simulink model "sixswitch"  (R2024b)
settings: Solver=ode23tb  StartTime=0.0  StopTime=1.0  MaxStep=sixswitch_maxstep  RelTol=1e-4
InitFcn:
  | p2s_dir = fileparts(get_param(bdroot, 'FileName'));
  | if ~isempty(p2s_dir), addpath(p2s_dir); end
  | clear p2s_dir
  | sixswitch_params;
values from neighbouring files (symbols this model uses):
  decouple_gain = 2*pi*fgrid*L    (= 0.125663706144)    [sixswitch_params.m]
  fgrid = 50    [sixswitch_params.m]
  fs = 100e3    (= 100000)    [sixswitch_params.m]
  grid_sr = 32e3    (= 32000)    [sixswitch_params.m]
  gridFrequency = 50    [sixswitch_params.m]
  id_ref_const = 13.8    [sixswitch_params.m]
  load_ramp_X0 = 100    [sixswitch_params.m]
  load_ramp_XFinal = 18000    [sixswitch_params.m]
  Pss = struct()    [sixswitch_params.m]
  vc_avg_T = (1/fs)*10    (= 0.0001)    [sixswitch_params.m]
  vd_dec_const = -10    [sixswitch_params.m]
  Vdc_ref = Vin    (= 700)    [sixswitch_params.m]
  Vgrid_pk = (gridVoltageLLrms/sqrt(3))*sqrt(2)    [sixswitch_params.m]
  vq_const = -1.85    [sixswitch_params.m]
undefined symbols (not defined in the file or in its folder): cc, pll, sixswitch_y0, vc
libraries: slpidlib x4
Description:
  | Ideal-switch translation of SixSwitch.plecs (see README.md)
settings Model: Creator=Jonathan  LastModifiedBy=Jonathan
settings SolverCC: ZeroCrossAlgorithm=Adaptive
settings DebuggingCC: MaxConsecutiveZCsMsg=none

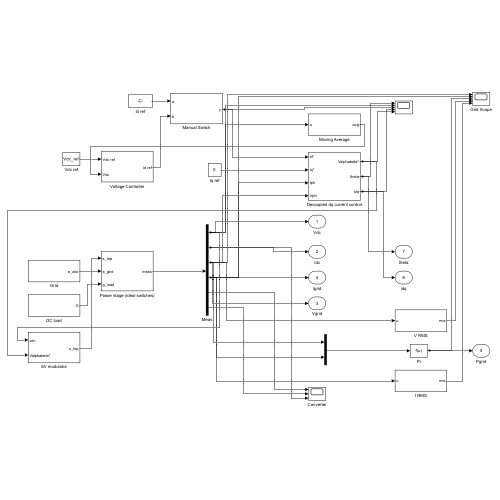
[thumbnail: Simulink's stored preview of the top-level diagram]
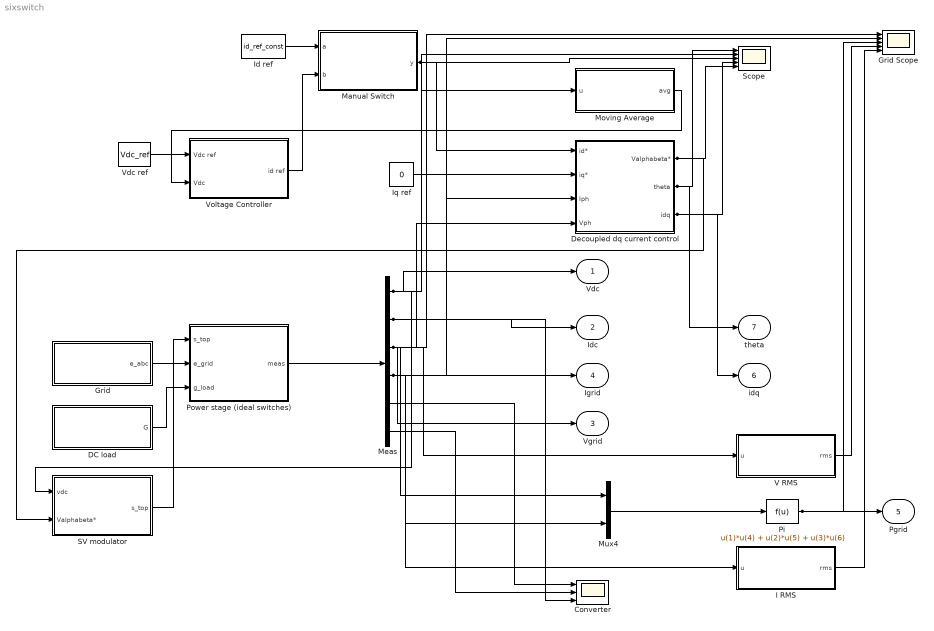
== system sixswitch ==
  Converter : Scope  NumInputPorts=3
  DC load : Subsystem
  Decoupled dq current control : Subsystem
  Grid : Subsystem
  Grid Scope : Scope  NumInputPorts=5
  I RMS : Subsystem
  Id ref : Constant  Value=id_ref_const
  Iq ref : Constant  Value=0
  Manual Switch : Subsystem
  Meas : Demux  Outputs=[1 1 3 3 3 3]
  Moving Average : Subsystem
  Mux4 : Mux  Inputs=2
  Pi : Fcn  Expr=u(1)*u(4) + u(2)*u(5) + u(3)*u(6)
  Power stage (ideal switches) : Subsystem
  SV modulator : Subsystem
  Scope : Scope  NumInputPorts=5
  V RMS : Subsystem
  Vdc ref : Constant  Value=Vdc_ref
  Voltage Controller : Subsystem
  Vdc : Outport
  Idc : Outport  Port=2
  Vgrid : Outport  Port=3
  Igrid : Outport  Port=4
  Pgrid : Outport  Port=5
  idq : Outport  Port=6
  theta : Outport  Port=7
  wires:
  Id ref/1 -> Manual Switch/1(a)
  Vdc ref/1 -> Voltage Controller/1(Vdc ref)
  Grid/1(e_abc) -> Power stage (ideal switches)/2(e_grid)
  DC load/1(G) -> Power stage (ideal switches)/3(g_load)
  Voltage Controller/1(id ref) -> Manual Switch/2(b)
  SV modulator/1(s_top) -> Power stage (ideal switches)/1(s_top)
  Power stage (ideal switches)/1(meas) -> Meas/1
  Manual Switch/1(y) -> Scope/3, Decoupled dq current control/1(id*)
  Iq ref/1 -> Decoupled dq current control/2(iq*)
  Decoupled dq current control/2(theta) -> Scope/1, theta/1
  Decoupled dq current control/1(Valphabeta*) -> SV modulator/2(Valphabeta*), Scope/5
  Meas/2 -> Converter/3, Idc/1
  Meas/1 -> Scope/2, Moving Average/1(u), SV modulator/1(vdc), Vdc/1
  Meas/3 -> V RMS/1(u), Decoupled dq current control/4(Vph), Mux4/1, Grid Scope/1, Vgrid/1
  Meas/4 -> Grid Scope/2, I RMS/1(u), Decoupled dq current control/3(Iph), Mux4/2, Igrid/1
  Meas/5 -> Converter/1
  Meas/6 -> Converter/2
  Moving Average/1(avg) -> Voltage Controller/2(Vdc)
  Decoupled dq current control/3(idq) -> Scope/4, idq/1
  Mux4/1 -> Pi/1
  V RMS/1(rms) -> Grid Scope/4
  Pi/1 -> Grid Scope/3, Pgrid/1
  I RMS/1(rms) -> Grid Scope/5

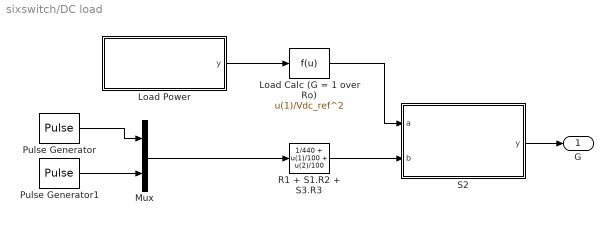
== system sixswitch/DC load ==
  Load Calc (G = 1 over Ro) : Fcn  Expr=u(1)/Vdc_ref^2
  Load Power : Subsystem
  Mux : Mux  Inputs=2
  Pulse Generator : DiscretePulseGenerator  PulseType=Time based  Period=0.02  PulseWidth=50  PhaseDelay=0.030
  Pulse Generator1 : DiscretePulseGenerator  PulseType=Time based  Period=0.01  PulseWidth=50  PhaseDelay=0.045
  R1 + S1.R2 + S3.R3 : Fcn  Expr=1/440 + u(1)/100 + u(2)/100
  S2 : Subsystem
  G : Outport
  wires:
  R1 + S1.R2 + S3.R3/1 -> S2/2(b)
  Mux/1 -> R1 + S1.R2 + S3.R3/1
  Pulse Generator/1 -> Mux/1
  Pulse Generator1/1 -> Mux/2
  Load Power/1(y) -> Load Calc (G = 1 over Ro)/1
  Load Calc (G = 1 over Ro)/1 -> S2/1(a)
  S2/1(y) -> G/1

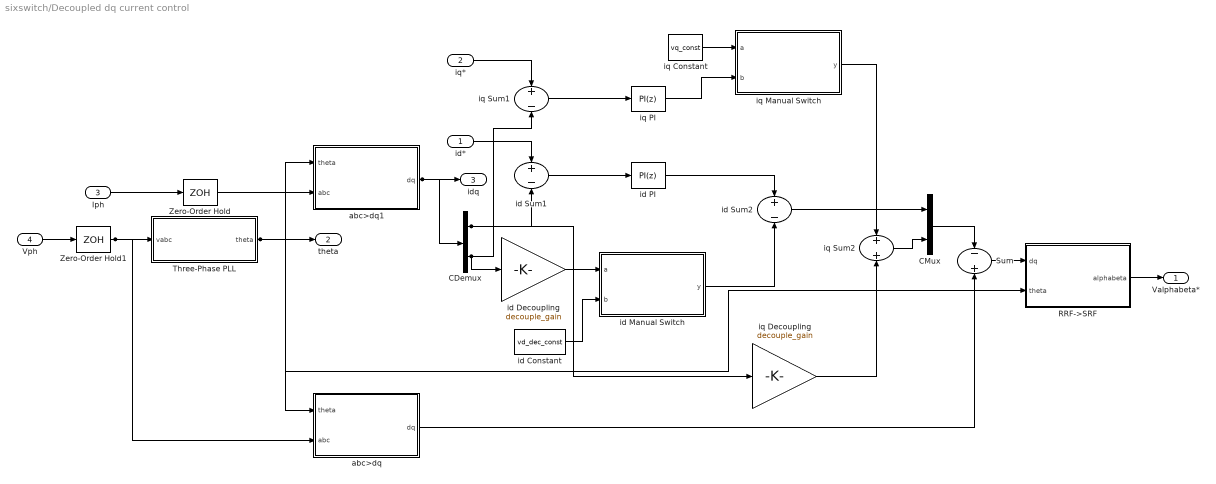
== system sixswitch/Decoupled dq current control ==
  id* : Inport
  iq* : Inport  Port=2
  Iph : Inport  Port=3
  Vph : Inport  Port=4
  CDemux : Demux  Outputs=2
  CMux : Mux  Inputs=2
  RRF->SRF : Subsystem
  Sum : Sum  Inputs=-+
  Three-Phase PLL : Subsystem
  Zero-Order Hold : ZeroOrderHold  SampleTime=1/grid_sr
  Zero-Order Hold1 : ZeroOrderHold  SampleTime=1/grid_sr
  abc>dq : Subsystem
  abc>dq1 : Subsystem
  id Constant : Constant  Value=vd_dec_const
  id Decoupling : Gain  Gain=decouple_gain
  id Manual Switch : Subsystem
  id PI : slpidlib/PID Controller  Controller=PI  Form=Parallel  TimeDomain=Discrete-time  UseExternalTs=off  SampleTime=cc.Ts  IntegratorMethod=Forward Euler  FilterMethod=Forward Euler  ControllerParametersSource=internal  P=cc.kp  I=cc.ki  UseKiTs=off  D=0  UseExternalDerivativeSource=off  N=100  UseFilter=on  TunerSelectOption=Transfer Function Based (PID Tuner App)  InitialConditionSource=internal  InitialConditionForIntegrator=0  InitialConditionForFilter=0  DifferentiatorICPrevScaledInput=0  ExternalReset=none  TrackingMode=off  Kt=1  LimitOutput=on  SatLimitsSource=internal  UpperSaturationLimit=cc.up  LowerSaturationLimit=cc.lo  LinearizeAsGain=off  AntiWindupMode=clamping  Kb=1  LimitIntegrator=off  UpperIntegratorSaturationLimit=inf  LowerIntegratorSaturationLimit=-inf  POutMin=[]  POutMax=[]  IOutMin=[]  IOutMax=[]  DOutMin=[]  DOutMax=[]  NOutMin=[]  NOutMax=[]  SumOutMin=[]  SumOutMax=[]  SaturationOutMin=[]  SaturationOutMax=[]  PParamMin=[]  PParamMax=[]  IParamMin=[]  IParamMax=[]  DParamMin=[]  DParamMax=[]  NParamMin=[]  NParamMax=[]  KbParamMin=[]  KbParamMax=[]  KtParamMin=[]  KtParamMax=[]  KbOutMin=[]  KbOutMax=[]  KtOutMin=[]  KtOutMax=[]  IntegratorOutMin=[]  IntegratorOutMax=[]  FilterOutMin=[]  FilterOutMax=[]  SumI1OutMin=[]  SumI1OutMax=[]  SumI2OutMin=[]  SumI2OutMax=[]  SumI3OutMin=[]  SumI3OutMax=[]  SumI4OutMin=[]  SumI4OutMax=[]  SumDOutMin=[]  SumDOutMax=[]  DifferentiatorOutMin=[]  DifferentiatorOutMax=[]  FilterDiffOutCoefMin=[]  FilterDiffOutCoefMax=[]  ReciprocalOutMin=[]  ReciprocalOutMax=[]  SumDenOutMin=[]  SumDenOutMax=[]  SumNumOutMin=[]  SumNumOutMax=[]  DivideOutMin=[]  DivideOutMax=[]  UdiffTsProdOutMin=[]  UdiffTsProdOutMax=[]  NTsProdOutMin=[]  NTsProdOutMax=[]  UintegralTsProdOutMin=[]  UintegralTsProdOutMax=[]  UngainTsProdOutMin=[]  UngainTsProdOutMax=[]  ClampingZeroOutDataTypeStr=Inherit: Inherit via back propagation  ClampingZeroOutMin=[]  ClampingZeroOutMax=[]  FilterDenConstantOutDataTypeStr=Inherit: Inherit via back propagation  FilterDenConstantOutMin=[]  FilterDenConstantOutMax=[]  PCopyOutDataTypeStr=Inherit: Inherit via back propagation  PCopyOutMin=[]  PCopyOutMax=[]  NCopyOutDataTypeStr=Inherit: Inherit via back propagation  NCopyOutMin=[]  NCopyOutMax=[]  IntegratorContinuousStateAttributes=''  IntegratorStateMustResolveToSignalObject=off  IntegratorRTWStateStorageClass=Auto  FilterContinuousStateAttributes=''  FilterStateMustResolveToSignalObject=off  FilterRTWStateStorageClass=Auto  ParallelPVariant=InternalParameters  IdealPVariant=Disabled  IVariant=InternalParameters  DVariant=Disabled  IntegratorVariant=Discrete  SatVariant=Enabled  AWVariant=DiscClampingParallel  PCopyVariant=Disabled  TRVariant=Disabled  FdbkBlocksVariant=Forward  IdealPFdbkVariant=Disabled  SatFdbkVariant=Disabled  DerivativeFilterVariant=Disabled  NVariant=Disabled  NCopyVariant=Disabled_SignalSpec  FilterICVariant=Disabled  IntegratorICVariant=InternalICs  ExternalResetVariant=Disabled  TRSumVariant=Passthrough  SumFdbkVariant=Disabled  SumVariant=Sum_PI  TsampFilterVariant=InternalTs  TsampNgainVariant=Passthrough  TsampIntegralVariant=Disabled_SignalSpec  ExternalSaturationOutDataTypeStr=Inherit: Same as second input  DerivativeSourceVariant=Disabled  PreIntVariant=InternalPreInt
      settings: LibrarySourceBlock=simulink/Discrete/Discrete PID Controller
  id Sum1 : Sum  Inputs=+-
  id Sum2 : Sum  Inputs=+-
  iq Constant : Constant  Value=vq_const
  iq Decoupling : Gain  Gain=decouple_gain
  iq Manual Switch : Subsystem
  iq PI : slpidlib/PID Controller  Controller=PI  Form=Parallel  TimeDomain=Discrete-time  UseExternalTs=off  SampleTime=cc.Ts  IntegratorMethod=Forward Euler  FilterMethod=Forward Euler  ControllerParametersSource=internal  P=cc.kp  I=cc.ki  UseKiTs=off  D=0  UseExternalDerivativeSource=off  N=100  UseFilter=on  TunerSelectOption=Transfer Function Based (PID Tuner App)  InitialConditionSource=internal  InitialConditionForIntegrator=0  InitialConditionForFilter=0  DifferentiatorICPrevScaledInput=0  ExternalReset=none  TrackingMode=off  Kt=1  LimitOutput=on  SatLimitsSource=internal  UpperSaturationLimit=cc.up  LowerSaturationLimit=cc.lo  LinearizeAsGain=off  AntiWindupMode=back-calculation  Kb=cc.kbc  LimitIntegrator=off  UpperIntegratorSaturationLimit=inf  LowerIntegratorSaturationLimit=-inf  POutMin=[]  POutMax=[]  IOutMin=[]  IOutMax=[]  DOutMin=[]  DOutMax=[]  NOutMin=[]  NOutMax=[]  SumOutMin=[]  SumOutMax=[]  SaturationOutMin=[]  SaturationOutMax=[]  PParamMin=[]  PParamMax=[]  IParamMin=[]  IParamMax=[]  DParamMin=[]  DParamMax=[]  NParamMin=[]  NParamMax=[]  KbParamMin=[]  KbParamMax=[]  KtParamMin=[]  KtParamMax=[]  KbOutMin=[]  KbOutMax=[]  KtOutMin=[]  KtOutMax=[]  IntegratorOutMin=[]  IntegratorOutMax=[]  FilterOutMin=[]  FilterOutMax=[]  SumI1OutMin=[]  SumI1OutMax=[]  SumI2OutMin=[]  SumI2OutMax=[]  SumI3OutMin=[]  SumI3OutMax=[]  SumI4OutMin=[]  SumI4OutMax=[]  SumDOutMin=[]  SumDOutMax=[]  DifferentiatorOutMin=[]  DifferentiatorOutMax=[]  FilterDiffOutCoefMin=[]  FilterDiffOutCoefMax=[]  ReciprocalOutMin=[]  ReciprocalOutMax=[]  SumDenOutMin=[]  SumDenOutMax=[]  SumNumOutMin=[]  SumNumOutMax=[]  DivideOutMin=[]  DivideOutMax=[]  UdiffTsProdOutMin=[]  UdiffTsProdOutMax=[]  NTsProdOutMin=[]  NTsProdOutMax=[]  UintegralTsProdOutMin=[]  UintegralTsProdOutMax=[]  UngainTsProdOutMin=[]  UngainTsProdOutMax=[]  ClampingZeroOutDataTypeStr=Inherit: Inherit via back propagation  ClampingZeroOutMin=[]  ClampingZeroOutMax=[]  FilterDenConstantOutDataTypeStr=Inherit: Inherit via back propagation  FilterDenConstantOutMin=[]  FilterDenConstantOutMax=[]  PCopyOutDataTypeStr=Inherit: Inherit via back propagation  PCopyOutMin=[]  PCopyOutMax=[]  NCopyOutDataTypeStr=Inherit: Inherit via back propagation  NCopyOutMin=[]  NCopyOutMax=[]  IntegratorContinuousStateAttributes=''  IntegratorStateMustResolveToSignalObject=off  IntegratorRTWStateStorageClass=Auto  FilterContinuousStateAttributes=''  FilterStateMustResolveToSignalObject=off  FilterRTWStateStorageClass=Auto  ParallelPVariant=InternalParameters  IdealPVariant=Disabled  IVariant=InternalParameters  DVariant=Disabled  IntegratorVariant=Discrete  SatVariant=Enabled  AWVariant=BackCalculation  PCopyVariant=Disabled  TRVariant=Disabled  FdbkBlocksVariant=Forward  IdealPFdbkVariant=Disabled  SatFdbkVariant=Disabled  DerivativeFilterVariant=Disabled  NVariant=Disabled  NCopyVariant=Disabled_SignalSpec  FilterICVariant=Disabled  IntegratorICVariant=InternalICs  ExternalResetVariant=Disabled  TRSumVariant=Passthrough  SumFdbkVariant=Disabled  SumVariant=Sum_PI  TsampFilterVariant=InternalTs  TsampNgainVariant=Passthrough  TsampIntegralVariant=Disabled_SignalSpec  ExternalSaturationOutDataTypeStr=Inherit: Same as second input  DerivativeSourceVariant=Disabled  PreIntVariant=InternalPreInt
      settings: LibrarySourceBlock=simulink/Discrete/Discrete PID Controller
  iq Sum1 : Sum  Inputs=+-
  iq Sum2 : Sum
  Valphabeta* : Outport
  theta : Outport  Port=2
  idq : Outport  Port=3
  wires:
  Vph/1 -> Zero-Order Hold1/1
  Iph/1 -> Zero-Order Hold/1
  Zero-Order Hold1/1 -> abc>dq/2(abc), Three-Phase PLL/1(vabc)
  CMux/1 -> Sum/1
  Zero-Order Hold/1 -> abc>dq1/2(abc)
  id Manual Switch/1(y) -> id Sum2/2
  iq*/1 -> iq Sum1/1
  Three-Phase PLL/1(theta) -> RRF->SRF/2(theta), abc>dq1/1(theta), theta/1, abc>dq/1(theta)
  abc>dq1/1(dq) -> CDemux/1, idq/1
  RRF->SRF/1(alphabeta) -> Valphabeta*/1
  abc>dq/1(dq) -> Sum/2
  id Constant/1 -> id Manual Switch/2(b)
  id Decoupling/1 -> id Manual Switch/1(a)
  id*/1 -> id Sum1/1
  CDemux/1 -> id Sum1/2, iq Decoupling/1
  id PI/1 -> id Sum2/1
  CDemux/2 -> iq Sum1/2, id Decoupling/1
  iq Sum1/1 -> iq PI/1
  id Sum1/1 -> id PI/1
  iq Decoupling/1 -> iq Sum2/2
  iq Constant/1 -> iq Manual Switch/1(a)
  iq PI/1 -> iq Manual Switch/2(b)
  iq Manual Switch/1(y) -> iq Sum2/1
  id Sum2/1 -> CMux/1
  iq Sum2/1 -> CMux/2
  Sum/1 -> RRF->SRF/1(dq)

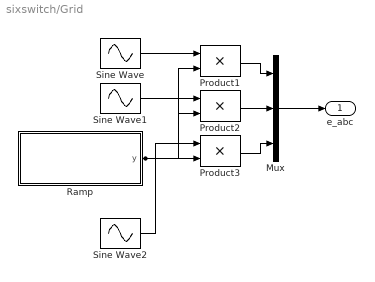
== system sixswitch/Grid ==
  Mux : Mux  Inputs=3
  Product1 : Product  Inputs=**
  Product2 : Product  Inputs=**
  Product3 : Product  Inputs=**
  Ramp : Subsystem
  Sine Wave : Sin  Amplitude=Vgrid_pk  Frequency=2*pi*gridFrequency  SampleTime=0
  Sine Wave1 : Sin  Amplitude=Vgrid_pk  Frequency=2*pi*gridFrequency  Phase=-2*pi/3  SampleTime=0
  Sine Wave2 : Sin  Amplitude=Vgrid_pk  Frequency=2*pi*gridFrequency  Phase=2*pi/3  SampleTime=0
  e_abc : Outport
  wires:
  Sine Wave/1 -> Product1/1
  Sine Wave1/1 -> Product2/1
  Product1/1 -> Mux/1
  Sine Wave2/1 -> Product3/1
  Ramp/1(y) -> Product1/2, Product2/2, Product3/2
  Product2/1 -> Mux/2
  Product3/1 -> Mux/3
  Mux/1 -> e_abc/1

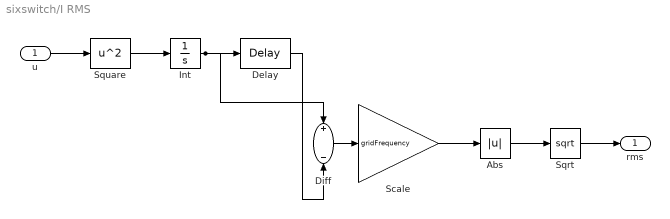
== system sixswitch/I RMS ==
  u : Inport
  Abs : Abs  SaturateOnIntegerOverflow=off
  Delay : TransportDelay  DelayTime=1/(gridFrequency)  BufferSize=131072
  Diff : Sum  Inputs=+-
  Int : Integrator
  Scale : Gain  Gain=gridFrequency
  Sqrt : Sqrt
  Square : Math  Operator=square
  rms : Outport
  wires:
  u/1 -> Square/1
  Int/1 -> Diff/1, Delay/1
  Square/1 -> Int/1
  Diff/1 -> Scale/1
  Delay/1 -> Diff/2
  Sqrt/1 -> rms/1
  Abs/1 -> Sqrt/1
  Scale/1 -> Abs/1

== system sixswitch/Manual Switch ==
  a : Inport
  b : Inport  Port=2
  Switch : Switch  Criteria=u2 > Threshold  Threshold=0.5  SaturateOnIntegerOverflow=off  InputSameDT=off
  sel : Constant  Value=double(sel_idref == 1)
  y : Outport
  wires:
  a/1 -> Switch/1
  sel/1 -> Switch/2
  b/1 -> Switch/3
  Switch/1 -> y/1

== system sixswitch/Moving Average ==
  u : Inport
  Delay : TransportDelay  DelayTime=vc_avg_T  BufferSize=131072
  Diff : Sum  Inputs=+-
  Int : Integrator
  Scale : Gain  Gain=1/(vc_avg_T)
  avg : Outport
  wires:
  u/1 -> Int/1
  Int/1 -> Diff/1, Delay/1
  Delay/1 -> Diff/2
  Scale/1 -> avg/1
  Diff/1 -> Scale/1

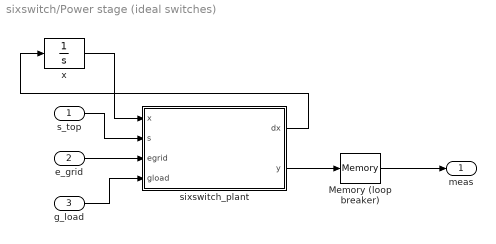
== system sixswitch/Power stage (ideal switches) ==
  s_top : Inport
  e_grid : Inport  Port=2
  g_load : Inport  Port=3
  Memory (loop breaker) : Memory  InitialCondition=sixswitch_y0
  sixswitch_plant : MATLAB Function  TreatAsAtomicUnit=on
  x : Integrator  InitialCondition=Pss.x0
  meas : Outport
  wires:
  x/1 -> sixswitch_plant/1(x)
  sixswitch_plant/2(y) -> Memory (loop breaker)/1
  sixswitch_plant/1(dx) -> x/1
  s_top/1 -> sixswitch_plant/2(s)
  e_grid/1 -> sixswitch_plant/3(egrid)
  g_load/1 -> sixswitch_plant/4(gload)
  Memory (loop breaker)/1 -> meas/1

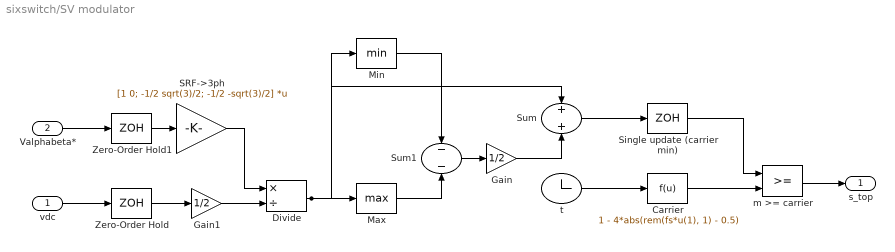
== system sixswitch/SV modulator ==
  vdc : Inport
  Valphabeta* : Inport  Port=2
  Carrier : Fcn  Expr=1 - 4*abs(rem(fs*u(1), 1) - 0.5)
  Divide : Product  Inputs=*/
  Gain : Gain  Gain=1/2
  Gain1 : Gain  Gain=1/2
  Max : MinMax  Function=max
  Min : MinMax
  SRF->3ph : Gain  Gain=[1 0; -1/2 sqrt(3)/2; -1/2 -sqrt(3)/2]  Multiplication=Matrix(K*u)
  Single update (carrier min) : ZeroOrderHold  SampleTime=1/fs
  Sum : Sum
  Sum1 : Sum  Inputs=--
  Zero-Order Hold : ZeroOrderHold  SampleTime=1/fs
  Zero-Order Hold1 : ZeroOrderHold  SampleTime=1/fs
  m >= carrier : RelationalOperator  OutDataTypeStr=boolean  RndMeth=Simplest  InputSameDT=off
  t : Clock
  s_top : Outport
  wires:
  vdc/1 -> Zero-Order Hold/1
  Valphabeta*/1 -> Zero-Order Hold1/1
  Zero-Order Hold/1 -> Gain1/1
  Zero-Order Hold1/1 -> SRF->3ph/1
  Gain1/1 -> Divide/2
  SRF->3ph/1 -> Divide/1
  Divide/1 -> Sum/1, Min/1, Max/1
  Min/1 -> Sum1/1
  Sum1/1 -> Gain/1
  Max/1 -> Sum1/2
  Sum/1 -> Single update (carrier min)/1
  Gain/1 -> Sum/2
  t/1 -> Carrier/1
  Single update (carrier min)/1 -> m >= carrier/1
  Carrier/1 -> m >= carrier/2
  m >= carrier/1 -> s_top/1

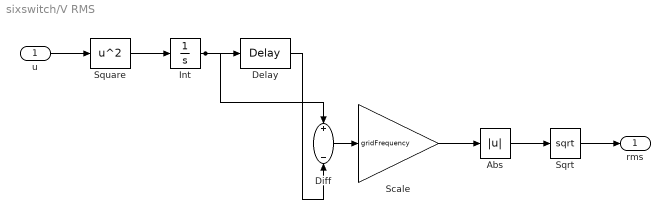
== system sixswitch/V RMS ==
  u : Inport
  Abs : Abs  SaturateOnIntegerOverflow=off
  Delay : TransportDelay  DelayTime=1/(gridFrequency)  BufferSize=131072
  Diff : Sum  Inputs=+-
  Int : Integrator
  Scale : Gain  Gain=gridFrequency
  Sqrt : Sqrt
  Square : Math  Operator=square
  rms : Outport
  wires:
  Square/1 -> Int/1
  u/1 -> Square/1
  Diff/1 -> Scale/1
  Delay/1 -> Diff/2
  Int/1 -> Diff/1, Delay/1
  Abs/1 -> Sqrt/1
  Scale/1 -> Abs/1
  Sqrt/1 -> rms/1

== system sixswitch/Voltage Controller ==
  Vdc ref : Inport
  Vdc : Inport  Port=2
  Discrete PID Controller : slpidlib/PID Controller  Controller=PI  Form=Parallel  TimeDomain=Discrete-time  UseExternalTs=off  SampleTime=vc.Ts  IntegratorMethod=Forward Euler  FilterMethod=Forward Euler  ControllerParametersSource=internal  P=vc.kp  I=vc.ki  UseKiTs=off  D=0  UseExternalDerivativeSource=off  N=100  UseFilter=on  TunerSelectOption=Transfer Function Based (PID Tuner App)  InitialConditionSource=internal  InitialConditionForIntegrator=0  InitialConditionForFilter=0  DifferentiatorICPrevScaledInput=0  ExternalReset=none  TrackingMode=off  Kt=1  LimitOutput=on  SatLimitsSource=internal  UpperSaturationLimit=vc.up  LowerSaturationLimit=vc.lo  LinearizeAsGain=off  AntiWindupMode=clamping  Kb=1  LimitIntegrator=off  UpperIntegratorSaturationLimit=inf  LowerIntegratorSaturationLimit=-inf  POutMin=[]  POutMax=[]  IOutMin=[]  IOutMax=[]  DOutMin=[]  DOutMax=[]  NOutMin=[]  NOutMax=[]  SumOutMin=[]  SumOutMax=[]  SaturationOutMin=[]  SaturationOutMax=[]  PParamMin=[]  PParamMax=[]  IParamMin=[]  IParamMax=[]  DParamMin=[]  DParamMax=[]  NParamMin=[]  NParamMax=[]  KbParamMin=[]  KbParamMax=[]  KtParamMin=[]  KtParamMax=[]  KbOutMin=[]  KbOutMax=[]  KtOutMin=[]  KtOutMax=[]  IntegratorOutMin=[]  IntegratorOutMax=[]  FilterOutMin=[]  FilterOutMax=[]  SumI1OutMin=[]  SumI1OutMax=[]  SumI2OutMin=[]  SumI2OutMax=[]  SumI3OutMin=[]  SumI3OutMax=[]  SumI4OutMin=[]  SumI4OutMax=[]  SumDOutMin=[]  SumDOutMax=[]  DifferentiatorOutMin=[]  DifferentiatorOutMax=[]  FilterDiffOutCoefMin=[]  FilterDiffOutCoefMax=[]  ReciprocalOutMin=[]  ReciprocalOutMax=[]  SumDenOutMin=[]  SumDenOutMax=[]  SumNumOutMin=[]  SumNumOutMax=[]  DivideOutMin=[]  DivideOutMax=[]  UdiffTsProdOutMin=[]  UdiffTsProdOutMax=[]  NTsProdOutMin=[]  NTsProdOutMax=[]  UintegralTsProdOutMin=[]  UintegralTsProdOutMax=[]  UngainTsProdOutMin=[]  UngainTsProdOutMax=[]  ClampingZeroOutDataTypeStr=Inherit: Inherit via back propagation  ClampingZeroOutMin=[]  ClampingZeroOutMax=[]  FilterDenConstantOutDataTypeStr=Inherit: Inherit via back propagation  FilterDenConstantOutMin=[]  FilterDenConstantOutMax=[]  PCopyOutDataTypeStr=Inherit: Inherit via back propagation  PCopyOutMin=[]  PCopyOutMax=[]  NCopyOutDataTypeStr=Inherit: Inherit via back propagation  NCopyOutMin=[]  NCopyOutMax=[]  IntegratorContinuousStateAttributes=''  IntegratorStateMustResolveToSignalObject=off  IntegratorRTWStateStorageClass=Auto  FilterContinuousStateAttributes=''  FilterStateMustResolveToSignalObject=off  FilterRTWStateStorageClass=Auto  ParallelPVariant=InternalParameters  IdealPVariant=Disabled  IVariant=InternalParameters  DVariant=Disabled  IntegratorVariant=Discrete  SatVariant=Enabled  AWVariant=DiscClampingParallel  PCopyVariant=Disabled  TRVariant=Disabled  FdbkBlocksVariant=Forward  IdealPFdbkVariant=Disabled  SatFdbkVariant=Disabled  DerivativeFilterVariant=Disabled  NVariant=Disabled  NCopyVariant=Disabled_SignalSpec  FilterICVariant=Disabled  IntegratorICVariant=InternalICs  ExternalResetVariant=Disabled  TRSumVariant=Passthrough  SumFdbkVariant=Disabled  SumVariant=Sum_PI  TsampFilterVariant=InternalTs  TsampNgainVariant=Passthrough  TsampIntegralVariant=Disabled_SignalSpec  ExternalSaturationOutDataTypeStr=Inherit: Same as second input  DerivativeSourceVariant=Disabled  PreIntVariant=InternalPreInt
      settings: LibrarySourceBlock=simulink/Discrete/Discrete PID Controller
  Sum1 : Sum  Inputs=+-
  id ref : Outport
  wires:
  Vdc ref/1 -> Sum1/1
  Vdc/1 -> Sum1/2
  Sum1/1 -> Discrete PID Controller/1
  Discrete PID Controller/1 -> id ref/1

== system sixswitch/DC load/Load Power ==
  Limit : Saturate  UpperLimit=max(load_ramp_X0,load_ramp_XFinal)  LowerLimit=min(load_ramp_X0,load_ramp_XFinal)
  Ramp : Fcn  Expr=(load_ramp_X0) + (load_ramp_slope)*(u(1)-(load_ramp_start))*(u(1)>(load_ramp_start))
  t : Clock
  y : Outport
  wires:
  t/1 -> Ramp/1
  Ramp/1 -> Limit/1
  Limit/1 -> y/1

== system sixswitch/DC load/S2 ==
  a : Inport
  b : Inport  Port=2
  Switch : Switch  Criteria=u2 > Threshold  Threshold=0.5  SaturateOnIntegerOverflow=off  InputSameDT=off
  sel : Constant  Value=double(sel_load == 2)
  y : Outport
  wires:
  a/1 -> Switch/1
  sel/1 -> Switch/2
  b/1 -> Switch/3
  Switch/1 -> y/1

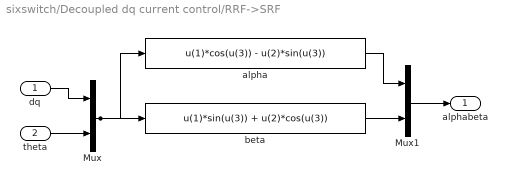
== system sixswitch/Decoupled dq current control/RRF->SRF ==
  dq : Inport
  theta : Inport  Port=2
  Mux : Mux  Inputs=2
  Mux1 : Mux  Inputs=2
  alpha : Fcn  Expr=u(1)*cos(u(3)) - u(2)*sin(u(3))
  beta : Fcn  Expr=u(1)*sin(u(3)) + u(2)*cos(u(3))
  alphabeta : Outport
  wires:
  dq/1 -> Mux/1
  theta/1 -> Mux/2
  alpha/1 -> Mux1/1
  Mux/1 -> alpha/1, beta/1
  Mux1/1 -> alphabeta/1
  beta/1 -> Mux1/2

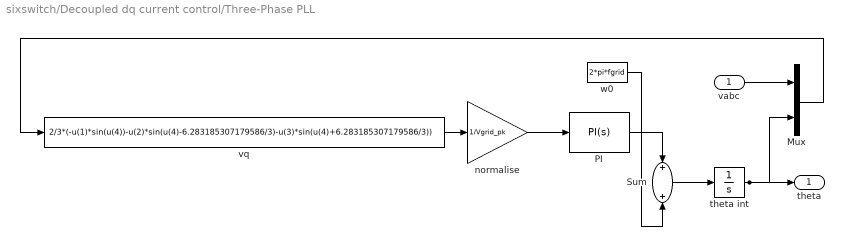
== system sixswitch/Decoupled dq current control/Three-Phase PLL ==
  vabc : Inport
  Mux : Mux  Inputs=2
  PI : slpidlib/PID Controller  Controller=PI  Form=Parallel  TimeDomain=Continuous-time  UseExternalTs=off  SampleTime=-1  IntegratorMethod=Forward Euler  FilterMethod=Forward Euler  ControllerParametersSource=internal  P=pll.kp  I=pll.ki  UseKiTs=off  D=0  UseExternalDerivativeSource=off  N=100  UseFilter=on  TunerSelectOption=Transfer Function Based (PID Tuner App)  InitialConditionSource=internal  InitialConditionForIntegrator=0  InitialConditionForFilter=0  DifferentiatorICPrevScaledInput=0  ExternalReset=none  TrackingMode=off  Kt=1  LimitOutput=off  SatLimitsSource=internal  UpperSaturationLimit=inf  LowerSaturationLimit=-inf  LinearizeAsGain=on  AntiWindupMode=none  Kb=1  LimitIntegrator=off  UpperIntegratorSaturationLimit=inf  LowerIntegratorSaturationLimit=-inf  POutMin=[]  POutMax=[]  IOutMin=[]  IOutMax=[]  DOutMin=[]  DOutMax=[]  NOutMin=[]  NOutMax=[]  SumOutMin=[]  SumOutMax=[]  SaturationOutMin=[]  SaturationOutMax=[]  PParamMin=[]  PParamMax=[]  IParamMin=[]  IParamMax=[]  DParamMin=[]  DParamMax=[]  NParamMin=[]  NParamMax=[]  KbParamMin=[]  KbParamMax=[]  KtParamMin=[]  KtParamMax=[]  KbOutMin=[]  KbOutMax=[]  KtOutMin=[]  KtOutMax=[]  IntegratorOutMin=[]  IntegratorOutMax=[]  FilterOutMin=[]  FilterOutMax=[]  SumI1OutMin=[]  SumI1OutMax=[]  SumI2OutMin=[]  SumI2OutMax=[]  SumI3OutMin=[]  SumI3OutMax=[]  SumI4OutMin=[]  SumI4OutMax=[]  SumDOutMin=[]  SumDOutMax=[]  DifferentiatorOutMin=[]  DifferentiatorOutMax=[]  FilterDiffOutCoefMin=[]  FilterDiffOutCoefMax=[]  ReciprocalOutMin=[]  ReciprocalOutMax=[]  SumDenOutMin=[]  SumDenOutMax=[]  SumNumOutMin=[]  SumNumOutMax=[]  DivideOutMin=[]  DivideOutMax=[]  UdiffTsProdOutMin=[]  UdiffTsProdOutMax=[]  NTsProdOutMin=[]  NTsProdOutMax=[]  UintegralTsProdOutMin=[]  UintegralTsProdOutMax=[]  UngainTsProdOutMin=[]  UngainTsProdOutMax=[]  ClampingZeroOutDataTypeStr=Inherit: Inherit via back propagation  ClampingZeroOutMin=[]  ClampingZeroOutMax=[]  FilterDenConstantOutDataTypeStr=Inherit: Inherit via back propagation  FilterDenConstantOutMin=[]  FilterDenConstantOutMax=[]  PCopyOutDataTypeStr=Inherit: Inherit via back propagation  PCopyOutMin=[]  PCopyOutMax=[]  NCopyOutDataTypeStr=Inherit: Inherit via back propagation  NCopyOutMin=[]  NCopyOutMax=[]  IntegratorContinuousStateAttributes=''  IntegratorStateMustResolveToSignalObject=off  IntegratorRTWStateStorageClass=Auto  FilterContinuousStateAttributes=''  FilterStateMustResolveToSignalObject=off  FilterRTWStateStorageClass=Auto  ParallelPVariant=InternalParameters  IdealPVariant=Disabled  IVariant=InternalParameters  DVariant=Disabled  IntegratorVariant=Continuous  SatVariant=Disabled  AWVariant=Passthrough  PCopyVariant=Disabled  TRVariant=Disabled  FdbkBlocksVariant=Forward  IdealPFdbkVariant=Disabled  SatFdbkVariant=Disabled  DerivativeFilterVariant=Disabled  NVariant=Disabled  NCopyVariant=Disabled_SignalSpec  FilterICVariant=Disabled  IntegratorICVariant=InternalICs  ExternalResetVariant=Disabled  TRSumVariant=Passthrough  SumFdbkVariant=Disabled  SumVariant=Sum_PI  TsampFilterVariant=InternalTs  TsampNgainVariant=Passthrough  TsampIntegralVariant=Disabled_SignalSpec  ExternalSaturationOutDataTypeStr=Inherit: Same as second input  DerivativeSourceVariant=Disabled  PreIntVariant=InternalPreInt
  Sum : Sum
  normalise : Gain  Gain=1/Vgrid_pk
  theta int : Integrator
  vq : Fcn  Expr=2/3*(-u(1)*sin(u(4))-u(2)*sin(u(4)-6.283185307179586/3)-u(3)*sin(u(4)+6.283185307179586/3))
  w0 : Constant  Value=2*pi*fgrid
  theta : Outport
  wires:
  normalise/1 -> PI/1
  vq/1 -> normalise/1
  theta int/1 -> Mux/2, theta/1
  Sum/1 -> theta int/1
  w0/1 -> Sum/2
  Mux/1 -> vq/1
  PI/1 -> Sum/1
  vabc/1 -> Mux/1

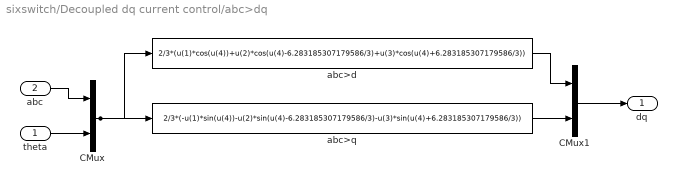
== system sixswitch/Decoupled dq current control/abc>dq ==
  theta : Inport
  abc : Inport  Port=2
  CMux : Mux  Inputs=2
  CMux1 : Mux  Inputs=2
  abc>d : Fcn  Expr=2/3*(u(1)*cos(u(4))+u(2)*cos(u(4)-6.283185307179586/3)+u(3)*cos(u(4)+6.283185307179586/3))
  abc>q : Fcn  Expr=2/3*(-u(1)*sin(u(4))-u(2)*sin(u(4)-6.283185307179586/3)-u(3)*sin(u(4)+6.283185307179586/3))
  dq : Outport
  wires:
  abc/1 -> CMux/1
  theta/1 -> CMux/2
  CMux/1 -> abc>d/1, abc>q/1
  CMux1/1 -> dq/1
  abc>q/1 -> CMux1/2
  abc>d/1 -> CMux1/1

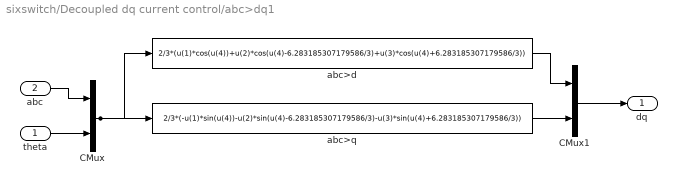
== system sixswitch/Decoupled dq current control/abc>dq1 ==
  theta : Inport
  abc : Inport  Port=2
  CMux : Mux  Inputs=2
  CMux1 : Mux  Inputs=2
  abc>d : Fcn  Expr=2/3*(u(1)*cos(u(4))+u(2)*cos(u(4)-6.283185307179586/3)+u(3)*cos(u(4)+6.283185307179586/3))
  abc>q : Fcn  Expr=2/3*(-u(1)*sin(u(4))-u(2)*sin(u(4)-6.283185307179586/3)-u(3)*sin(u(4)+6.283185307179586/3))
  dq : Outport
  wires:
  theta/1 -> CMux/2
  abc/1 -> CMux/1
  CMux/1 -> abc>d/1, abc>q/1
  CMux1/1 -> dq/1
  abc>q/1 -> CMux1/2
  abc>d/1 -> CMux1/1

== system sixswitch/Decoupled dq current control/id Manual Switch ==
  a : Inport
  b : Inport  Port=2
  Switch : Switch  Criteria=u2 > Threshold  Threshold=0.5  SaturateOnIntegerOverflow=off  InputSameDT=off
  sel : Constant  Value=double(sel_dec_d == 1)
  y : Outport
  wires:
  a/1 -> Switch/1
  b/1 -> Switch/3
  sel/1 -> Switch/2
  Switch/1 -> y/1

== system sixswitch/Decoupled dq current control/iq Manual Switch ==
  a : Inport
  b : Inport  Port=2
  Switch : Switch  Criteria=u2 > Threshold  Threshold=0.5  SaturateOnIntegerOverflow=off  InputSameDT=off
  sel : Constant  Value=double(sel_q == 1)
  y : Outport
  wires:
  b/1 -> Switch/3
  a/1 -> Switch/1
  Switch/1 -> y/1
  sel/1 -> Switch/2

== system sixswitch/Grid/Ramp ==
  Limit : Saturate  UpperLimit=max(0,1)  LowerLimit=min(0,1)
  Ramp : Fcn  Expr=(0) + (grid_ramp_slope)*(u(1)-(grid_ramp_start))*(u(1)>(grid_ramp_start))
  t : Clock
  y : Outport
  wires:
  t/1 -> Ramp/1
  Ramp/1 -> Limit/1
  Limit/1 -> y/1

== matlab function sixswitch/Power stage (ideal switches)/sixswitch_plant ==
  data: dx output; x input; y output; s input; egrid input; gload input; Pss parameter
function [dx, y] = sixswitch_plant(x, s, egrid, gload, Pss)
%SIXSWITCH_PLANT  Ideal-switch power stage of "SixSwitch.plecs" (body of a MATLAB Function block).
%
% Three-phase two-level converter ("2-Level MOSFET Conv.", dead time "off" in the PLECS model)
% on a DC link C1 (60 uF behind 4.2 mOhm) with a resistive DC load. AC side per phase:
%
%   leg --L (400 uH, "Inductor")--X--Lf (35 uH, "Filter")--+--Rg (0.4)--e_grid--N
%                                 |
%                                 Rd (4.7) -- Cf (2.2 uF) -- N
%
% The DC side floats with respect to the grid neutral N, so the converter-side currents sum
% to zero and the common-mode voltage follows from that constraint. The 0.4 uH in series with
% each damping resistor is neglected. MOSFETs are ideal switches (no dead time, so the top
% gate alone sets each leg).
%
% States  x = [iL(3); ig(3); vC(3); vC1]
%   iL  converter-side inductor currents, positive from node X into the converter leg
%   ig  grid-side currents, positive from the grid into node X (the direction measured by
%       the "3ph Meter" that feeds the current controller)
%   vC  filter capacitor voltages, vC1 DC-link capacitor voltage
% Inputs
%   s      3 top-gate signals (1 = leg tied to DC+)
%   egrid  3 grid source voltages (V)
%   gload  DC load conductance (S)
% Outputs
%   y = [Vdc; Idc_load; Vgrid(3) (meter voltages to N); Igrid(3); iL(3); vX(3)]
%#codegen

P = Pss;   % parameter struct from the workspace

iL = x(1:3);
ig = x(4:6);
vC = x(7:9);
vC1 = x(10);
sd = double(s);

iconv = sum(sd .* iL);                                  % current into DC+ from the converter
vdc = (vC1 + P.Resr * iconv) / (1 + P.Resr * gload);
iload = gload * vdc;

vX = vC + P.Rd * (ig - iL);                             % filter node voltage to N
vk = sd * vdc;                                          % leg voltages to DC-
v0N = (sum(vX) - sum(vk)) / 3;                          % DC- potential relative to N

dx = zeros(10, 1);
dx(1:3) = (vX - vk - v0N) / P.L;
dx(4:6) = (egrid - P.Rg * ig - vX) / P.Lf;
dx(7:9) = (ig - iL) / P.Cf;
dx(10) = (iconv - iload) / P.C1;

vmeter = egrid - P.Rg * ig;
y = [vdc; iload; vmeter; ig; iL; vX];
end
